simulink model "si_hmm_mismatch_supervisor"  (R2025b)
settings: Solver=FixedStepDiscrete  StartTime=0.0  StopTime=119.80000000000001  FixedStep=0.20000000000000001  RelTol=1e-3
model workspace (MAT data in the model file):
  a = 0.985815842352
  p.transition = [0.973416289593  0.0220588235294  0.00452488687783; 0.0374862183021  0.930540242558  0.03197353914; 0.0222929936306  0.0859872611465  0.891719745223]
  p.emission = [0.757166947723  0.238336143901  0.00449690837549; 0.185104052574  0.702081051479  0.112814895947; 0.00630914826498  0.1261829653  0.867507886435]
  p.initial = [0.782608695652 0.173913043478 0.0434782608696]
  p.dt = 0.2
  p.bias = [-0.000531055568177; 0.0549490044319; 0.135060369474]
  p.cutpoints = [0.025 0.095]
  p.nominal_tau = 10
  p.kp = 2
  p.ki = 0.2
  p.actuator_bias = 0.35
  p.supervised = 1
  reference_data = [0 0.2 0.4 0.6 0.8 1 1.2 1.4 1.6 1.8 2 2.2 ... (1200 elements, 600x2)]
  sensor_error = [0 0.2 0.4 0.6 0.8 1 1.2 1.4 1.6 1.8 2 2.2 ... (1200 elements, 600x2)]
settings Model: Creator=runner  LastModifiedBy=runner

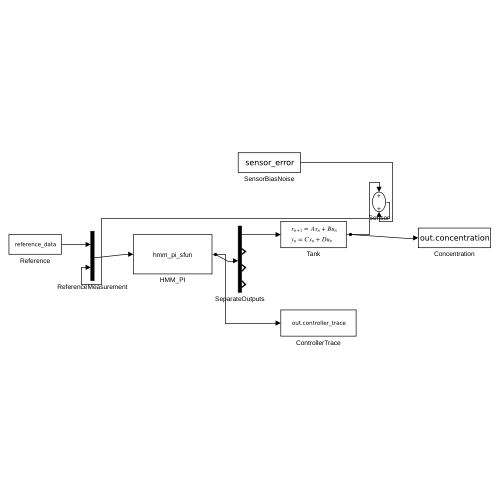
[thumbnail: Simulink's stored preview of the top-level diagram]
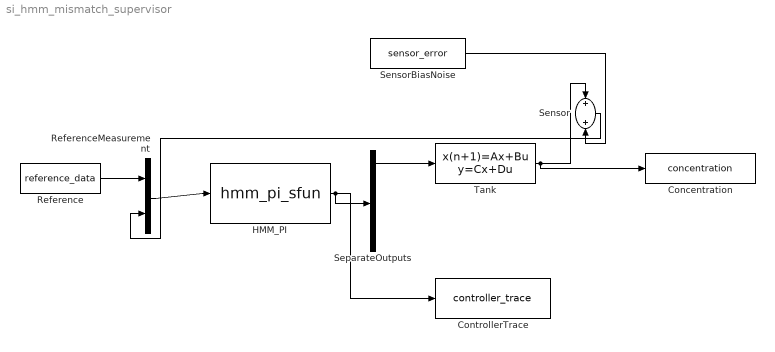
== system si_hmm_mismatch_supervisor ==
  Concentration : ToWorkspace  VariableName=concentration  SaveFormat=Structure With Time  SampleTime=-1
  ControllerTrace : ToWorkspace  VariableName=controller_trace  SaveFormat=Structure With Time  SampleTime=-1
  HMM_PI : S-Function  FunctionName=hmm_pi_sfun  Parameters=p  SFunctionDeploymentMode=off  EnableBusSupport=off
  Reference : FromWorkspace  VariableName=reference_data  SampleTime=p.dt  Interpolate=off  OutputAfterFinalValue=Holding final value
  ReferenceMeasurement : Mux  Inputs=2
  Sensor : Sum
  SensorBiasNoise : FromWorkspace  VariableName=sensor_error  SampleTime=p.dt  Interpolate=off  OutputAfterFinalValue=Holding final value
  SeparateOutputs : Demux  Outputs=[1 3 1 1]
  Tank : DiscreteStateSpace  A=a  B=1-a  D=0  InitialCondition=.35  SampleTime=0.2
  wires:
  Reference/1 -> ReferenceMeasurement/1
  Sensor/1 -> ReferenceMeasurement/2
  ReferenceMeasurement/1 -> HMM_PI/1
  HMM_PI/1 -> SeparateOutputs/1, ControllerTrace/1
  SeparateOutputs/1 -> Tank/1
  Tank/1 -> Concentration/1, Sensor/1
  SensorBiasNoise/1 -> Sensor/2
